simulink model "FSI09_1"  (R2024b)
settings: Solver=FixedStepAuto  StartTime=0.0  StopTime=t_stop  FixedStep=Ts  RelTol=1e-3
values from neighbouring files (symbols this model uses):
  b = 350    [FSI03WS.m]    (also in FSI04WS.m = 5; FSI08WS.m = 1.25663706144; FSI09WS.m = 3.14159265359)
  F = 1    [FSI08WS.m]    (also in FSI09WS.m = 10)
  f = chirp_end:(chirp_start/(length(t)-1)):chirp_start    [FSI04WS.m]    (also in FSI08WS.m = 5; FSI09WS.m = 5)
  v0 = 25    [FSI01WS.m]    (also in FSI08WS.m = 0; FSI09WS.m = 0)
libraries: fl_lib x8, nesl_utility x4
settings Model: Creator=fmiro  LastModifiedBy=fmiro

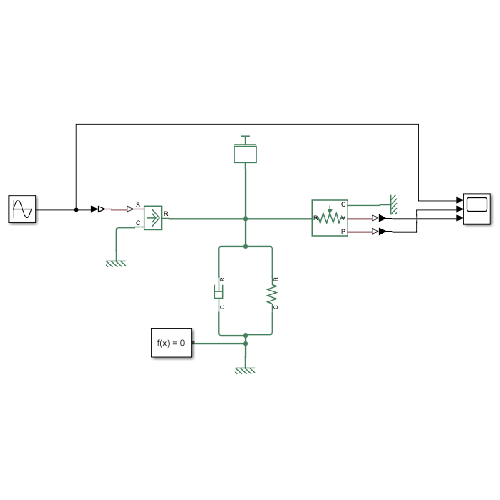
[thumbnail: Simulink's stored preview of the top-level diagram]
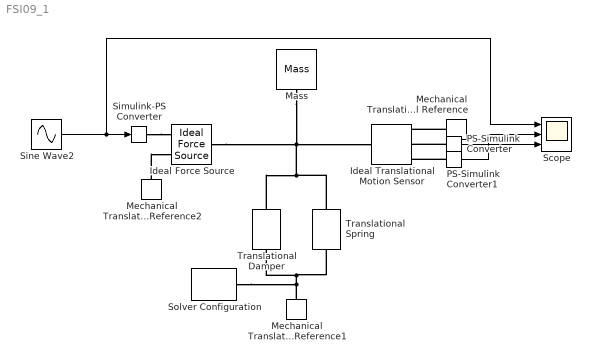
== system FSI09_1 ==
  Ideal Force Source : fl_lib/Mechanical/Mechanical Sources/Ideal Force Source
  Ideal Translational Motion Sensor : fl_lib/Mechanical/Mechanical Sensors/Ideal Translational Motion Sensor  reference=foundation.enum.MeasurementReference.difference  acceleration_port=false  velocity_port=true  position_port=true  offset=0 m
  Mass : fl_lib/Mechanical/Translational Elements/Mass  mass=m kg  num_ports=foundation.enum.numPorts2.one  v_specify=on  v_priority=High  v=v0 m/s  v_nominal_specify=off  v_nominal_value=1  v_nominal_unit=m/s  f_specify=off  f_priority=None  f=0 N  f_nominal_specify=off  f_nominal_value=1  f_nominal_unit=N
  Mechanical Translational Reference : fl_lib/Mechanical/Translational Elements/Mechanical Translational Reference
  Mechanical Translational Reference1 : fl_lib/Mechanical/Translational Elements/Mechanical Translational Reference
  Mechanical Translational Reference2 : fl_lib/Mechanical/Translational Elements/Mechanical Translational Reference
  PS-Simulink Converter : nesl_utility/PS-Simulink Converter  PhysicalDomain=network_engine_domain  SubClassName=ps_output  LeftPortType=input  RightPortType=output  PseudoPeriodic=off  Frequencies=[]  VectorFormat=inherit  Unit=inherit  AffineConversion=off
  PS-Simulink Converter1 : nesl_utility/PS-Simulink Converter  PhysicalDomain=network_engine_domain  SubClassName=ps_output  LeftPortType=input  RightPortType=output  PseudoPeriodic=off  Frequencies=[]  VectorFormat=inherit  Unit=inherit  AffineConversion=off
  Scope : Scope  NumInputPorts=3
  Simulink-PS Converter : nesl_utility/Simulink-PS Converter  PhysicalDomain=network_engine_domain  SubClassName=ps_input  LeftPortType=input  RightPortType=output  PseudoPeriodic=off  Frequencies=[]  NoiseDistribution=none  NoiseParameters=[]  Unit=1  AffineConversion=off  FilteringAndDerivatives=provide  SimscapeFilterOrder=1  InputFilterTimeConstant=0.001  UdotUserProvided=0
  Sine Wave2 : Sin  Amplitude=F  Frequency=2*pi*f  SampleTime=0
  Solver Configuration : nesl_utility/Solver Configuration  PhysicalDomain=network_engine_domain  SubClassName=solver  LeftPortType=input  RightPortType=generic  Tones=[]  Harmonics=[]  SimulateNoise=off  Profile=off  UseLocalSampling=off  EnableSwitchedLinearOptims=on  FrequencyDomain=off  UseCCode=off  RelTol=0.001  AbsTol=0.001  MinStep=1e-09  ToWorkspace=off  RevertToSquareIcSolve=off  NumHomotopyIterations=100  PhasorMode=off  PhasorModeNumHarmonics=1  ConsistencySolver=NEWTON_XTOL_AFTER_FTOL  IndexReductionMethod=DerivativeReplacement  DoDC=off  ResidualTolerance=1e-09  ConsistencyTolSource=GLOBAL  ConsistencyAbsTol=0.001  ConsistencyRelTol=0.001  ConsistencyTolFactor=0.001  UseLocalSolver=off  LocalSolverChoice=NE_BACKWARD_EULER_ADVANCER  ResolveIndetEquations=on  FunctionEvalNumThread=1  LocalSolverSampleTime=0.001  DoFixedCost=off  MaxNonlinIter=3  MaxModeIter=2  ComputeImpulses=off  ImpulseIterations=2  LinearAlgebra=auto  LinearAlgebraNumThread=0  EquationFormulation=NE_TIME_EF  DelaysMemoryBudget=1024  AutomaticFiltering=on  FilteringTimeConstant=0.001  PartitionStorageMethod=AS_NEEDED  PartitionMemoryBudget=1024  PartitionMethod=ROBUST  MultibodyUseLocalSolver=off  MultibodyLocalSolverChoice=ODE1  MultibodyLocalSolverSampleTime=0.001
  Translational Damper : fl_lib/Mechanical/Translational Elements/Translational Damper  D=b N*s/m  v_specify=off  v_priority=High  v=v0 m/s  v_nominal_specify=off  v_nominal_value=1  v_nominal_unit=m/s  f_specify=off  f_priority=None  f=0 N  f_nominal_specify=off  f_nominal_value=1  f_nominal_unit=N
  Translational Spring : fl_lib/Mechanical/Translational Elements/Translational Spring  spr_rate=k N/m  v_specify=off  v_priority=None  v=-v0 m/s  v_nominal_specify=off  v_nominal_value=1  v_nominal_unit=m/s  f_specify=off  f_priority=None  f=0 N  f_nominal_specify=off  f_nominal_value=1  f_nominal_unit=N  x_specify=on  x_priority=High  x=x0 m  x_nominal_specify=off  x_nominal_value=1  x_nominal_unit=m
  wires:
  Sine Wave2/1 -> Scope/1, Simulink-PS Converter/1
  PS-Simulink Converter1/1 -> Scope/2
  PS-Simulink Converter/1 -> Scope/3
  connections:
  Translational Damper/LConn1 -- Translational Spring/LConn1 -- Mass/LConn1 -- Ideal Force Source/LConn1 -- Ideal Translational Motion Sensor/LConn1
  Mechanical Translational Reference1/LConn1 -- Solver Configuration/RConn1 -- Translational Damper/RConn1 -- Translational Spring/RConn1
  Simulink-PS Converter/RConn1 -- Ideal Force Source/RConn1
  Mechanical Translational Reference2/LConn1 -- Ideal Force Source/RConn2
  Mechanical Translational Reference/LConn1 -- Ideal Translational Motion Sensor/RConn1
  PS-Simulink Converter/LConn1 -- Ideal Translational Motion Sensor/RConn2
  PS-Simulink Converter1/LConn1 -- Ideal Translational Motion Sensor/RConn3
